simulink model "ploop_test_4iv"  (R2025b)
settings: Solver=ode15s  StartTime=0.0  StopTime=1.5  RelTol=1e-3  EnableMultiTasking=on
libraries: roblocks x1
settings Model: Creator=pic  LastModifiedBy=ekkar
settings SolverCC: AlgebraicLoopSolver=TrustRegion
settings DataIOCC: SaveFormat=Array  SignalLoggingSaveFormat=ModelDataLogs  TimeSaveName=t  OutputSaveName=y  OutputOption=SpecifiedOutputTimes  OutputTimes=[0:0.001:1]'
settings OptimizationCC: ExpressionDepthLimit=2147483647.0  LifeSpan=inf
settings DebuggingCC: UnderspecifiedInitializationDetection=Classic  MergeDetectMultiDrivingBlocksExec=none  SolverPrmCheckMsg=warning  UnconnectedInputMsg=warning  UnconnectedOutputMsg=warning  UnconnectedLineMsg=warning  AllowSymbolicDim=off  StateNameClashWarn=warning  SFUnexpectedBacktrackingDiag=warning  SFNoUnconditionalDefaultTransitionDiag=warning  SFExecutionAtInitializationDiag=none  ArithmeticOperatorsInVariantConditions=warning
settings HardwareCC: ProdBitPerPointer=32.0  ProdBitPerSizeT=32.0  ProdBitPerPtrDiffT=32.0  ProdLargestAtomicFloat=None  ProdIntDivRoundTo=Undefined  ProdEndianess=Unspecified  ProdWordSize=32.0  ProdHWDeviceType=32-bit Generic
settings ModelReferenceCC: EnableRefExpFcnMdlSchedulingChecks=on  PropagateSignalLabelsOutOfModel=off
settings SFSimCC: SimUseLocalCustomCode=off  CustomCodeUndefinedFunction=UseInterfaceOnly
settings RTWCC: RTWUseLocalCustomCode=off  GPUComputeCapability=3.5
settings CodeAppCC: StateflowObjectComments=on
settings GRTTargetCC: TargetLangStandard=C89/C90 (ANSI)  CombineOutputUpdateFcns=off  GRTInterface=on
settings ConfigComp: CovMetricSettings=dw  CovSaveCumulativeToWorkspaceVar=on  CovSaveSingleToWorkspaceVar=on  CovExternalEMLEnable=off  CovSFcnEnable=off

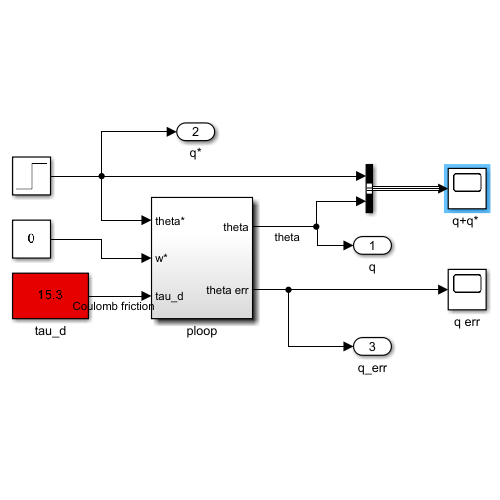
[thumbnail: Simulink's stored preview of the top-level diagram]
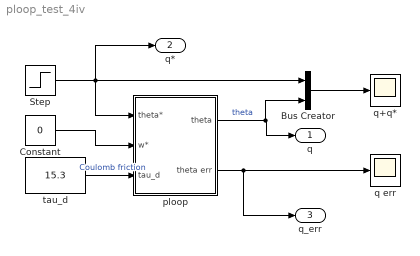
== system ploop_test_4iv ==
  Bus Creator : BusCreator  Inputs=2
  Constant : Constant  Value=0
  Step : Step  Time=0.1  After=0.1  SampleTime=0
  ploop : Subsystem
  q err : Scope
      settings: ActiveDisplayYMinimum=-0.0062499947781171194  ActiveDisplayYMaximum=0.05624995300305409  YLabel=theta error (rad)
  "q+q* " : Scope
      settings: ActiveDisplayYMinimum=-0.012983860488065279  ActiveDisplayYMaximum=0.1125537622764517  YLabel=theta (rad)
  tau_d : Constant  Value=15.3
  q : Outport  VectorParamsAs1DForOutWhenUnconnected=off
  q* : Outport  Port=2  VectorParamsAs1DForOutWhenUnconnected=off
  q_err : Outport  Port=3  VectorParamsAs1DForOutWhenUnconnected=off
  wires:
  ploop/1(theta) -> Bus Creator/2, q/1  "theta"
  ploop/2(theta err) -> q_err/1, q err/1
  tau_d/1 -> ploop/3(tau_d)  "Coulomb friction"
  Bus Creator/1 -> "q+q* "/1
  Constant/1 -> ploop/2(w*)
  Step/1 -> ploop/1(theta*), q*/1, Bus Creator/1

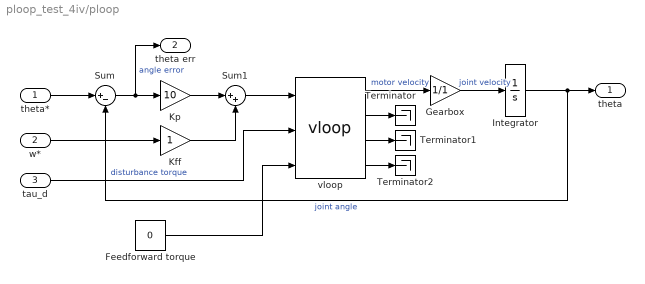
== system ploop_test_4iv/ploop ==
  theta* : Inport
  w* : Inport  Port=2
  tau_d : Inport  Port=3
  Feedforward torque : Constant  Value=0
  Gearbox : Gain  Gain=1/1
  Integrator : Integrator
  Kff : Gain
  Kp : Gain  Gain=10
  Sum : Sum  Inputs=|+-
  Sum1 : Sum  Inputs=|++
  Terminator : Terminator
  Terminator1 : Terminator
  Terminator2 : Terminator
  vloop : roblocks/Arm/vloop  J=39.3671  B=11.96  Km=1  tau_max=1e4  Kv=1562.7  Ki=15750  T=0.001
  theta : Outport  VectorParamsAs1DForOutWhenUnconnected=off
  theta err : Outport  Port=2  VectorParamsAs1DForOutWhenUnconnected=off
  wires:
  Sum/1 -> Kp/1, theta err/1  "angle error"
  Integrator/1 -> theta/1, Sum/2  "joint angle"
  theta*/1 -> Sum/1
  Kp/1 -> Sum1/1
  Sum1/1 -> vloop/1
  w*/1 -> Kff/1
  Kff/1 -> Sum1/2
  vloop/2 -> Terminator/1
  vloop/3 -> Terminator1/1
  vloop/4 -> Terminator2/1
  vloop/1 -> Gearbox/1  "motor velocity"
  tau_d/1 -> vloop/2  "disturbance torque"
  Feedforward torque/1 -> vloop/3
  Gearbox/1 -> Integrator/1  "joint velocity"
